simulink model "Quadrotor_6DoF"  (R2024a)
settings: Solver=ode45  StartTime=0.0  StopTime=50  MaxStep=0.01  RelTol=1e-3
values from neighbouring files (symbols this model uses):
  B_eff = [ kf,     kf,     kf,     kf ... (first row only)    [init_6dof_params.m]
  B_mixer = inv(B_eff)    [init_6dof_params.m]
  D_drag = diag([0.0, 0.0, 0.0])    [init_6dof_params.m]
  g = 9.81    [init_6dof_params.m]
  Kd_phi = 0.2142    [init_6dof_params.m]
  Kd_psi = 0.2880    (= 0.288)    [init_6dof_params.m]
  Kd_theta = 0.2142    [init_6dof_params.m]
  Kd_z = 10.8    [init_6dof_params.m]
  kf = (CT * rho * D_prop^4) / (4 * pi^2)    (= 1.4207049827e-05)    [init_6dof_params.m]
  km = (CQ * rho * D_prop^5) / (4 * pi^2)    (= 2.95248326405e-07)    [init_6dof_params.m]
  Kp_phi = 0.756    [init_6dof_params.m]
  Kp_psi = 0.640    (= 0.64)    [init_6dof_params.m]
  Kp_theta = 0.756    [init_6dof_params.m]
  Kp_z = 18.0    (= 18)    [init_6dof_params.m]
  m = 2.00    (= 2)    [init_6dof_params.m]    (also in run_step5_tests.m = masses(i); run_step7_px4_replay.m)
  omega_max_sq = omega_max^2    (= 888264.396098)    [init_6dof_params.m]
  test_case = 1    [init_6dof_params.m]    (also in run_step5_tests.m; run_step7_px4_replay.m = 7)
libraries: shared6dof x1
settings Model: SimulationMode=accelerator  SnapshotBufferSize=25  SnapshotInterval=25  Creator=tlnar  LastModifiedBy=tlnar

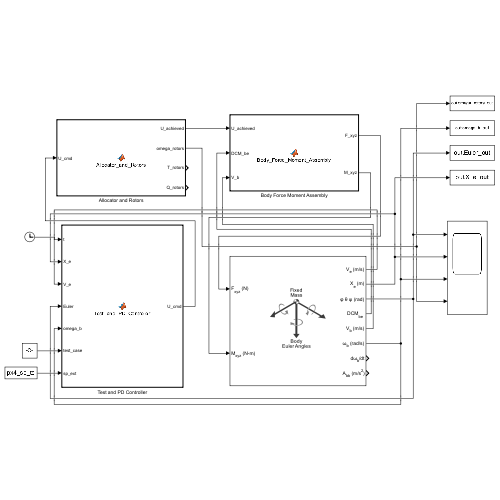
[thumbnail: Simulink's stored preview of the top-level diagram]
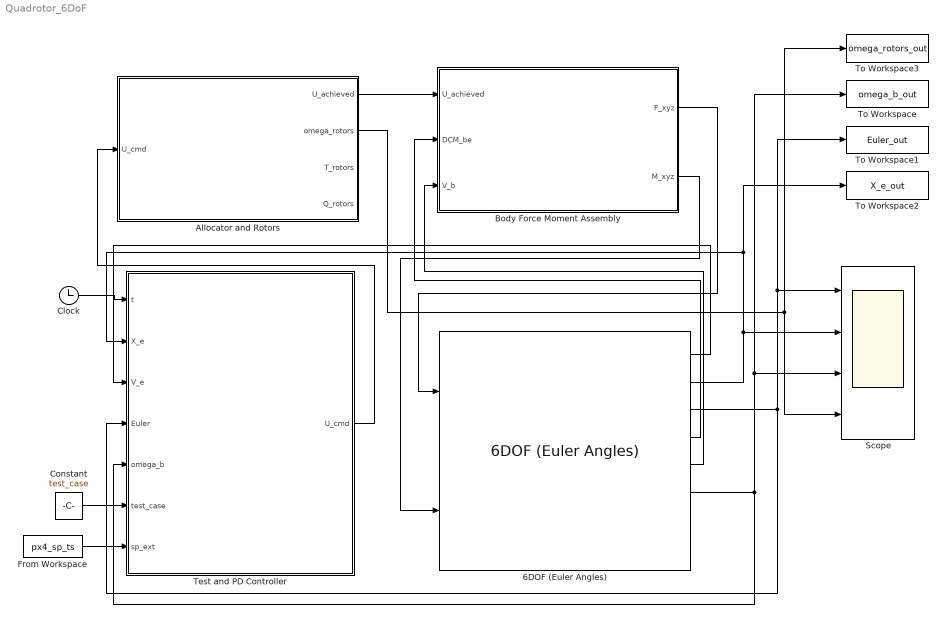
== system Quadrotor_6DoF ==
  6DOF (Euler Angles) : shared6dof/6DOF (Euler Angles)  units=Metric (MKS)  mtype=Fixed  rep=Euler Angles  xme_0=[0 0 -10]  Vm_0=[0 0 0]  eul_0=[0 0 0]  pm_0=[0 0 0]  mass_0=m  mass_e=0.5  mass_f=2.0  inertia=J  inertia_e=eye(3)  inertia_f=2*eye(3)  k_quat=1.0  vre_flag=on  abi_flag=off  aMode=0  xme_statename=''  Vm_statename=''  eul_statename=''  quat_statename=''  pm_statename=''  mass_statename=''
  Allocator and Rotors : MATLAB Function  TreatAsAtomicUnit=on
  Body Force Moment Assembly : MATLAB Function  TreatAsAtomicUnit=on
  Clock : Clock
  Constant : Constant  Value=test_case
  From Workspace : FromWorkspace  VariableName=px4_sp_ts
  Scope : Scope  NumInputPorts=4
  Test and PD Controller : MATLAB Function  TreatAsAtomicUnit=on
  To Workspace : ToWorkspace  VariableName=omega_b_out  SaveFormat=Timeseries  SampleTime=-1
  To Workspace1 : ToWorkspace  VariableName=Euler_out  SaveFormat=Timeseries  SampleTime=-1
  To Workspace2 : ToWorkspace  VariableName=X_e_out  SaveFormat=Timeseries  SampleTime=-1
  To Workspace3 : ToWorkspace  VariableName=omega_rotors_out  SaveFormat=Timeseries  SampleTime=-1
  wires:
  Test and PD Controller/1(U_cmd) -> Allocator and Rotors/1(U_cmd)
  Allocator and Rotors/1(U_achieved) -> Body Force Moment Assembly/1(U_achieved)
  Body Force Moment Assembly/1(F_xyz) -> 6DOF (Euler Angles)/1
  Body Force Moment Assembly/2(M_xyz) -> 6DOF (Euler Angles)/2
  6DOF (Euler Angles)/4 -> Body Force Moment Assembly/2(DCM_be)
  6DOF (Euler Angles)/5 -> Body Force Moment Assembly/3(V_b)
  6DOF (Euler Angles)/2 -> Scope/2, To Workspace2/1, Test and PD Controller/2(X_e)
  6DOF (Euler Angles)/1 -> Test and PD Controller/3(V_e)
  6DOF (Euler Angles)/3 -> To Workspace1/1, Scope/1, Test and PD Controller/4(Euler)
  6DOF (Euler Angles)/6 -> Test and PD Controller/5(omega_b), To Workspace/1, Scope/3
  Clock/1 -> Test and PD Controller/1(t)
  Allocator and Rotors/2(omega_rotors) -> To Workspace3/1, Scope/4
  Constant/1 -> Test and PD Controller/6(test_case)
  From Workspace/1 -> Test and PD Controller/7(sp_ext)

== matlab function Quadrotor_6DoF/Test and PD Controller ==
  data: t input; X_e input; V_e input; Euler input; omega_b input; test_case input; sp_ext input; U_cmd output; m parameter; g parameter; Kp_z parameter; Kd_z parameter; Kp_phi parameter; Kd_phi parameter; Kp_theta parameter; Kd_theta parameter; Kp_psi parameter; Kd_psi parameter
function U_cmd = Test_and_PD_Controller(t, X_e, V_e, Euler, omega_b, test_case, sp_ext, ...
    m, g, Kp_z, Kd_z, Kp_phi, Kd_phi, Kp_theta, Kd_theta, Kp_psi, Kd_psi)

phi   = Euler(1);
theta = Euler(2);
psi   = Euler(3);

p = omega_b(1);
q = omega_b(2);
r = omega_b(3);

% Convert NED down-position & down-velocity to positive-up altitude
z_alt     = -X_e(3);
z_dot_alt = -V_e(3);

U1        = m * g;
tau_phi   = 0.0;
tau_theta = 0.0;
tau_psi   = 0.0;

switch test_case
    case 1  % Test 1: Open-Loop Hover Equilibrium
        U1 = m * g;

    case 21 % Test 2a: Pure Roll Pulse
        U1 = m * g;
        if t >= 0.5 && t < 0.7
            tau_phi = 0.01;
        end

    case 22 % Test 2b: Pure Pitch Pulse
        U1 = m * g;
        if t >= 0.5 && t < 0.7
            tau_theta = 0.01;
        end

    case 3  % Test 3: Pure Yaw Pulse
        U1 = m * g;
        if t >= 1.0 && t < 2.0
            tau_psi = 0.02;
        end

    case 4  % Test 4: Payload Equilibrium
        U1 = m * g;

    case 5  % Test 5: Closed-Loop PD Attitude Step (10 deg at t = 1.0 s)
        z_ref = 10.0;
        if t >= 1.0
            phi_ref   = deg2rad(10);
            theta_ref = deg2rad(10);
        else
            phi_ref   = 0.0;
            theta_ref = 0.0;
        end
        psi_ref = 0.0;

        cos_tilt  = max(0.5, cos(phi) * cos(theta));
        U1        = (m * g + Kp_z * (z_ref - z_alt) - Kd_z * z_dot_alt) / cos_tilt;
        e_psi     = atan2(sin(psi_ref - psi), cos(psi_ref - psi));
        tau_phi   = Kp_phi   * (phi_ref   - phi)   - Kd_phi   * p;
        tau_theta = Kp_theta * (theta_ref - theta) - Kd_theta * q;
        tau_psi   = Kp_psi   * e_psi               - Kd_psi   * r;

    case 7  % Step 7: External PX4 SITL Attitude Setpoint Replay
        z_ref     = 10.0;
        phi_ref   = sp_ext(1);
        theta_ref = sp_ext(2);
        psi_ref   = sp_ext(3);

        cos_tilt  = max(0.5, cos(phi) * cos(theta));
        U1        = (m * g + Kp_z * (z_ref - z_alt) - Kd_z * z_dot_alt) / cos_tilt;
        e_psi     = atan2(sin(psi_ref - psi), cos(psi_ref - psi));
        tau_phi   = Kp_phi   * (phi_ref   - phi)   - Kd_phi   * p;
        tau_theta = Kp_theta * (theta_ref - theta) - Kd_theta * q;
        tau_psi   = Kp_psi   * e_psi               - Kd_psi   * r;
end

U_cmd = [U1; tau_phi; tau_theta; tau_psi];
end

== matlab function Quadrotor_6DoF/Body Force Moment Assembly ==
  data: U_achieved input; F_xyz output; DCM_be input; V_b input; M_xyz output; D_drag parameter; m parameter; g parameter
function [F_xyz, M_xyz] = Body_Force_Moment_Assembly(U_achieved, DCM_be, V_b, D_drag, m, g)
% Extract achieved total thrust magnitude and moments
U1_ach    = U_achieved(1);
M_xyz     = U_achieved(2:4); % [tau_phi; tau_theta; tau_psi] about CoM in FRD [N*m]

% 1. Rotor thrust in FRD body frame (+Z_b is down, so thrust is -Z_b)
F_rotor_b = [0; 0; -U1_ach];

% 2. Gravity vector transformed from NED Earth frame [0; 0; m*g] to FRD body frame
F_gravity_b = DCM_be * [0; 0; m * g];

% 3. Linear body-axis aerodynamic drag
F_drag_b = -D_drag * V_b;

% 4. Resultant applied force at Center of Mass in FRD body axes [N]
F_xyz = F_rotor_b + F_gravity_b + F_drag_b;
end

== matlab function Quadrotor_6DoF/Allocator and Rotors ==
  data: U_cmd input; U_achieved output; omega_rotors output; T_rotors output; Q_rotors output; B_mixer parameter; B_eff parameter; kf parameter; km parameter; omega_max_sq parameter
function [U_achieved, omega_rotors, T_rotors, Q_rotors] = Allocator_and_Rotors(U_cmd, B_mixer, B_eff, kf, km, omega_max_sq)
% 1. Map virtual wrench U_cmd = [U1; tau_phi; tau_theta; tau_psi] to squared speeds
omega_sq_cmd = B_mixer * U_cmd;

% 2. Saturate squared rotor speeds within physical limits [0, omega_max^2]
omega_sq_sat = max(0, min(omega_max_sq, omega_sq_cmd));

% 3. Actual rotor angular speeds [rad/s]
omega_rotors = sqrt(omega_sq_sat);

% 4. Individual static rotor thrusts and reaction torques
T_rotors = kf * omega_sq_sat;
Q_rotors = km * omega_sq_sat;

% 5. Reconstruct actual achieved wrench [U1_ach; tau_phi_ach; tau_theta_ach; tau_psi_ach]
U_achieved = B_eff * omega_sq_sat;
end
